simulink model "DisplayDriver"  (R2024a)
settings: Solver=FixedStepDiscrete  StartTime=0.0  StopTime=10  FixedStep=0.01  RelTol=1e-3
model workspace (MAT data in the model file):
  DisplayRefresh_cycles = Simulink.Parameter
  DisplayRefresh_cycles.Value = 100
  DisplayRefresh_cycles.Complexity = 'real'
  DisplayRefresh_cycles.Dimensions = [1 1]
  DisplayRefresh_cycles.DataType = 'uint16'
  DisplayRetry_cycles = Simulink.Parameter
  DisplayRetry_cycles.Value = 50
  DisplayRetry_cycles.Complexity = 'real'
  DisplayRetry_cycles.Dimensions = [1 1]
  DisplayRetry_cycles.DataType = 'uint16'
values from neighbouring files (symbols this model uses):
  DisplayRefresh_cycles = 100    [DisplayDriver_data.m]
  DisplayRetry_cycles = 50    [DisplayDriver_data.m]
Description:
  | Anzeige: 4 Ziffern des 7-Segment-Moduls (I2C 0x71), ein Byte je Schreibauftrag
settings Model: ParameterArgumentNames=DisplayRefresh_cycles,DisplayRetry_cycles  Creator=danie  LastModifiedBy=danie
settings OptimizationCC: DefaultParameterBehavior=Inlined  EnhancedBackFolding=on  PassReuseOutputArgsAs=Individual arguments  ZeroExternalMemoryAtStartup=off  ZeroInternalMemoryAtStartup=off  OptimizeBlockOrder=speed  DifferentSizesBufferReuse=on  OptimizationCustomize=off  EfficientTunableParamExpr=on
settings DebuggingCC: ParameterTunabilityLossMsg=error
settings HardwareCC: ProdBitPerPointer=32  ProdBitPerSizeT=32  ProdBitPerPtrDiffT=32  ProdLargestAtomicInteger=Long  ProdLargestAtomicFloat=Double  ProdWordSize=32  ProdLongLongMode=on  ProdHWDeviceType=ARM Compatible->ARM Cortex-M
settings SFSimCC: MATLABDynamicMemAlloc=off
settings RTWCC: Description=AUTOSAR  SystemTargetFile=autosar.tlc  GenCodeOnly=on  GenerateMakefile=off  TemplateMakefile=ert_default_tmf  DataTypeReplacement=CDataTypesFixedWidth
settings CodeAppCC: ForceParamTrailComments=on  IgnoreCustomStorageClasses=off  MaxIdLength=63  OperatorAnnotations=on  SimulinkDataObjDesc=on  SFDataObjDesc=on  InsertBlockDesc=on
settings STFCustomTargetCC: MultiwordLength=256  ParMdlRefBuildCompliant=on  CompOptLevelCompliant=on  IncludeMdlTerminateFcn=off  CombineOutputUpdateFcns=on  SuppressErrorStatus=on  ERTCustomFileBanners=on  SupportNonFinite=off  SupportComplex=off  SupportContinuousTime=off  SupportNonInlinedSFcns=off  RemoveResetFunc=on  MATLABClassNameForMDSCustomization=Simulink.SoftwareTarget.ERTCustomization  AutosarCompliant=on  GRTInterface=off  LookupTableObjectStructAxisOrder=2,1,3,4,...  LUTObjectStructOrderEvenSpacing=Size,Table,Breakpoints  SystemTargetFile=autosar.tlc
settings ERTTargetCC: TargetLangStandard=C99 (ISO)  ConcurrentExecutionCompliant=off  IncludeMdlTerminateFcn=off  SuppressErrorStatus=on  SupportNonFinite=off  SupportComplex=off  ModelStepFunctionPrototypeControlCompliant=off  CPPClassGenCompliant=off  AutosarCompliant=on  LookupTableObjectStructAxisOrder=2,1,3,4,...  LUTObjectStructOrderEvenSpacing=Size,Table,Breakpoints  InlinedParameterPlacement=NonHierarchical  ERTCustomFileTemplate=example_file_process.tlc  BooleanTrueId=TRUE  BooleanFalseId=FALSE

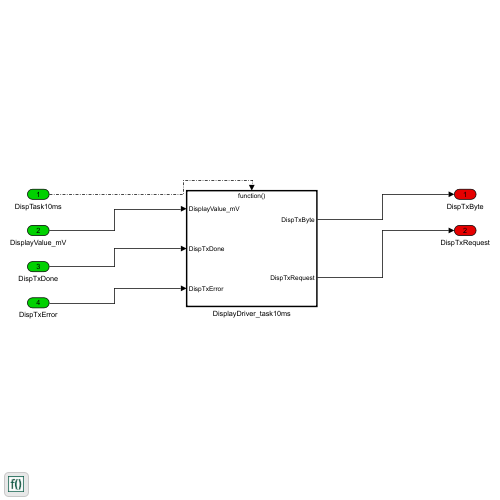
[thumbnail: Simulink's stored preview of the top-level diagram]
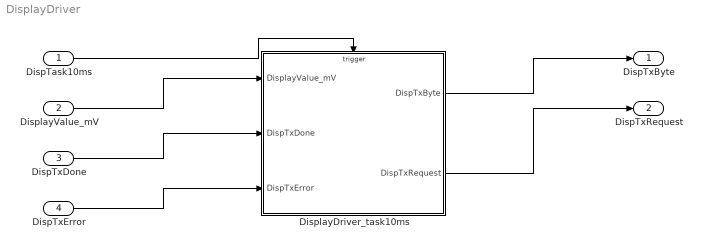
== system DisplayDriver ==
  DispTask10ms : Inport  SampleTime=0.01  OutputFunctionCall=on
  DisplayValue_mV : Inport  Port=2  OutDataTypeStr=uint16  PortDimensions=1
  DispTxDone : Inport  Port=3  OutDataTypeStr=uint8  PortDimensions=1
  DispTxError : Inport  Port=4  OutDataTypeStr=boolean  PortDimensions=1
  DisplayDriver_task10ms : Subsystem  TreatAsAtomicUnit=on
  DispTxByte : Outport  OutDataTypeStr=uint8  PortDimensions=1
  DispTxRequest : Outport  Port=2  OutDataTypeStr=uint8  PortDimensions=1
  wires:
  DispTask10ms/1 -> DisplayDriver_task10ms/Trigger
  DisplayValue_mV/1 -> DisplayDriver_task10ms/1(DisplayValue_mV)
  DispTxDone/1 -> DisplayDriver_task10ms/2(DispTxDone)
  DispTxError/1 -> DisplayDriver_task10ms/3(DispTxError)
  DisplayDriver_task10ms/1(DispTxByte) -> DispTxByte/1
  DisplayDriver_task10ms/2(DispTxRequest) -> DispTxRequest/1

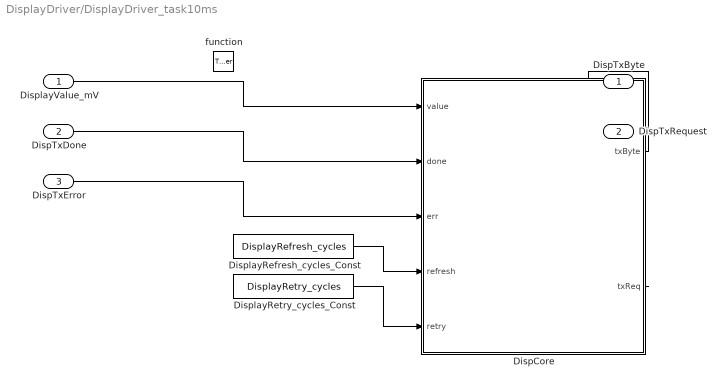
== system DisplayDriver/DisplayDriver_task10ms ==
  DisplayValue_mV : Inport
  DispTxDone : Inport  Port=2
  DispTxError : Inport  Port=3
  function : TriggerPort  TriggerType=function-call  VariantControl=(inherit)  SampleTimeType=periodic  SampleTime=0.01
  DispCore : MATLAB Function  TreatAsAtomicUnit=on
  DisplayRefresh_cycles_Const : Constant  Value=DisplayRefresh_cycles  OutDataTypeStr=uint16
  DisplayRetry_cycles_Const : Constant  Value=DisplayRetry_cycles  OutDataTypeStr=uint16
  DispTxByte : Outport
  DispTxRequest : Outport  Port=2
  wires:
  DisplayValue_mV/1 -> DispCore/1(value)
  DispTxDone/1 -> DispCore/2(done)
  DispTxError/1 -> DispCore/3(err)
  DisplayRefresh_cycles_Const/1 -> DispCore/4(refresh)
  DisplayRetry_cycles_Const/1 -> DispCore/5(retry)
  DispCore/1(txByte) -> DispTxByte/1
  DispCore/2(txReq) -> DispTxRequest/1

== matlab function DisplayDriver/DisplayDriver_task10ms/DispCore ==
  data: value input; txByte output; done input; err input; refresh input; retry input; txReq output
function [txByte, txReq] = DispCore(value, done, err, refresh, retry)
%DISPCORE Byte sequence for the 7-segment module (see DisplayDriver_create.m).
%#codegen
persistent req outByte step len frame shown age wait needClear inflight
if isempty(req)
    req = uint8(0);
    outByte = uint8(0);
    step = uint8(0);
    len = uint8(0);
    frame = zeros(15, 1, 'uint8');
    shown = uint16(65535);
    age = uint16(0);
    wait = uint16(0);
    needClear = true;
    inflight = false;
end
% result of the order in flight
if inflight && (done == req)
    inflight = false;
    if err
        step = uint8(0);
        needClear = true;
        shown = uint16(65535);
        wait = retry;
    end
end
if wait > uint16(0)
    wait = wait - uint16(1);
end
if age < uint16(65535)
    age = age + uint16(1);
end
if (~inflight) && (wait == uint16(0))
    if step == uint8(0)
        v = min(value, uint16(9999));
        if needClear || (v ~= shown) || (age >= refresh)
            n = uint8(0);
            if needClear
                n = uint8(1);
                frame(1) = uint8(118);   % 0x76 clear
            end
            digits = [idivide(v, uint16(1000)), mod(idivide(v, uint16(100)), uint16(10)), ...
                      mod(idivide(v, uint16(10)), uint16(10)), mod(v, uint16(10))];
            for k = 1:4
                frame(n + 1) = uint8(121);            % 0x79 cursor
                frame(n + 2) = uint8(k - 1);          % position
                frame(n + 3) = uint8(digits(k));      % digit
                n = n + uint8(3);
            end
            frame(n + 1) = uint8(119);                % 0x77 decimal points
            frame(n + 2) = uint8(1);                  % mask: point behind the first digit
            len = n + uint8(2);
            step = uint8(1);
            shown = v;
        end
    end
    if step > uint8(0)
        outByte = frame(step);
        if req == uint8(255)               % the counter wraps (I2cByteWriter): saturating at 255 stopped all orders
            req = uint8(0);
        else
            req = req + uint8(1);
        end
        inflight = true;
        if step == len
            step = uint8(0);
            age = uint16(0);
            needClear = false;
        else
            step = step + uint8(1);
        end
    end
end
txByte = outByte;
txReq = req;
